simulink model "ps_model"  (R2025b)
settings: Solver=ode23tb  StartTime=0.0  StopTime=simlength  FixedStep=tc  MaxStep=tc
values from neighbouring files (symbols this model uses):
  omega_grid_emulator_nom = w_grid    (= 314.159265359)    [grid_emulator.m]
  omega_grid_nom = w_grid    (= 314.159265359)    [grid_emulator.m]
  ugrid_factor = 1    [grid_emulator.m]
  V_phase_normalization_factor = Vgrid_phase_normalization_factor    [grid_emulator.m]
  Vdc_base = 720    [grid_emulator.m]
  vn_eta_pu = 0    [grid_emulator.m]
  vn_xi_pu = 0    [grid_emulator.m]
  vp_xi_pu = 1    [grid_emulator.m]
undefined symbols (not defined in the file or in its folder): CFi, fnom, fPWM_INV, i_nom, ki_i, ki_u, kp_i, kp_u, Ld2_trafo_out, magnitude, n10, number_of_cells, omega_nom, Q, q1Kalman, q2Kalman, q3Kalman, R_RLload, Rd2_trafo_out, rKalman, tc, time_load_step, ts_afe, ts_inv, tsample, u_nom, Vdc_nom
libraries: fl_lib x120, nesl_utility x67, ee_lib x7, cstblocks x4, moving_average_filter x4, single_phase_transformer_lib x3, lithium_ion_cell_lib x1, simulink x1, threephase_inductor_lib x1
(part 2 of 4)

== system ps_model/inverter/3ph_Dyn_simscape ==
  Electrical Reference1 : fl_lib/Electrical/Electrical Elements/Electrical Reference
  ph1 : single_phase_transformer_lib/single phase transformer  Lm=Lmu2_trafo_out H  n1=sqrt(3)/0.8  n2=1  Rd1=Rd2_trafo_out/2 Ohm  Rd2=Rd2_trafo_out/2 Ohm  Ld1=Ld2_trafo_out/2 H  Ld2=Ld2_trafo_out/2 H  Rfe=Rm2_trafo_out Ohm  phi_specify=off  phi_priority=None  phi=0 V*s  phi_nominal_specify=off  phi_nominal_value=1  phi_nominal_unit=V*s  i1_specify=off  i1_priority=None  i1=0 A  i1_nominal_specify=off  i1_nominal_value=1  i1_nominal_unit=A  i2_specify=off  i2_priority=None  i2=0 A  i2_nominal_specify=off  i2_nominal_value=1  i2_nominal_unit=A  ife_specify=off  ife_priority=None  ife=0 A  ife_nominal_specify=off  ife_nominal_value=1  ife_nominal_unit=A  u1_specify=off  u1_priority=None  u1=0 V  u1_nominal_specify=off  u1_nominal_value=1  u1_nominal_unit=V  u2_specify=off  u2_priority=None  u2=0 V  u2_nominal_specify=off  u2_nominal_value=1  u2_nominal_unit=V
      settings: InternalSimscapePortConfiguration="{\"Bottom\":[],\"Left\":[{\"id\":\"u1_p\",\"label\":\"u1(+)\",\"type\":\"foundation.electrical.electrical\"},{\"id\":\"u1_n\",\"label\":\"u1(-)\",\"type\":\"foundation.electrical.electrical\"}],\"Right\":[{\"id\":\"u2_p\",\"label\":\"u2(+)\",\"type\":\"foundation.electrical.electrical\"},{\"id\":\"u2_n\",\"label\":\"u2(-)\",\"type\":\"foundation.electrical.electrical\"}],\"Top\":[]}"
  ph2 : single_phase_transformer_lib/single phase transformer  Lm=Lmu2_trafo_out H  n1=sqrt(3)/0.8  n2=1  Rd1=Rd2_trafo_out/2 Ohm  Rd2=Rd2_trafo_out/2 Ohm  Ld1=Ld2_trafo_out/2 H  Ld2=Ld2_trafo_out/2 H  Rfe=Rm2_trafo_out Ohm  phi_specify=off  phi_priority=None  phi=0 V*s  phi_nominal_specify=off  phi_nominal_value=1  phi_nominal_unit=V*s  i1_specify=off  i1_priority=None  i1=0 A  i1_nominal_specify=off  i1_nominal_value=1  i1_nominal_unit=A  i2_specify=off  i2_priority=None  i2=0 A  i2_nominal_specify=off  i2_nominal_value=1  i2_nominal_unit=A  ife_specify=off  ife_priority=None  ife=0 A  ife_nominal_specify=off  ife_nominal_value=1  ife_nominal_unit=A  u1_specify=off  u1_priority=None  u1=0 V  u1_nominal_specify=off  u1_nominal_value=1  u1_nominal_unit=V  u2_specify=off  u2_priority=None  u2=0 V  u2_nominal_specify=off  u2_nominal_value=1  u2_nominal_unit=V
      settings: InternalSimscapePortConfiguration="{\"Bottom\":[],\"Left\":[{\"id\":\"u1_p\",\"label\":\"u1(+)\",\"type\":\"foundation.electrical.electrical\"},{\"id\":\"u1_n\",\"label\":\"u1(-)\",\"type\":\"foundation.electrical.electrical\"}],\"Right\":[{\"id\":\"u2_p\",\"label\":\"u2(+)\",\"type\":\"foundation.electrical.electrical\"},{\"id\":\"u2_n\",\"label\":\"u2(-)\",\"type\":\"foundation.electrical.electrical\"}],\"Top\":[]}"
  ph3 : single_phase_transformer_lib/single phase transformer  Lm=Lmu2_trafo_out H  n1=sqrt(3)/0.8  n2=1  Rd1=Rd2_trafo_out/2 Ohm  Rd2=Rd2_trafo_out/2 Ohm  Ld1=Ld2_trafo_out/2 H  Ld2=Ld2_trafo_out/2 H  Rfe=Rm2_trafo_out Ohm  phi_specify=off  phi_priority=None  phi=0 V*s  phi_nominal_specify=off  phi_nominal_value=1  phi_nominal_unit=V*s  i1_specify=off  i1_priority=None  i1=0 A  i1_nominal_specify=off  i1_nominal_value=1  i1_nominal_unit=A  i2_specify=off  i2_priority=None  i2=0 A  i2_nominal_specify=off  i2_nominal_value=1  i2_nominal_unit=A  ife_specify=off  ife_priority=None  ife=0 A  ife_nominal_specify=off  ife_nominal_value=1  ife_nominal_unit=A  u1_specify=off  u1_priority=None  u1=0 V  u1_nominal_specify=off  u1_nominal_value=1  u1_nominal_unit=V  u2_specify=off  u2_priority=None  u2=0 V  u2_nominal_specify=off  u2_nominal_value=1  u2_nominal_unit=V
      settings: InternalSimscapePortConfiguration="{\"Bottom\":[],\"Left\":[{\"id\":\"u1_p\",\"label\":\"u1(+)\",\"type\":\"foundation.electrical.electrical\"},{\"id\":\"u1_n\",\"label\":\"u1(-)\",\"type\":\"foundation.electrical.electrical\"}],\"Right\":[{\"id\":\"u2_p\",\"label\":\"u2(+)\",\"type\":\"foundation.electrical.electrical\"},{\"id\":\"u2_n\",\"label\":\"u2(-)\",\"type\":\"foundation.electrical.electrical\"}],\"Top\":[]}"
  ua : PMIOPort  Side=Right
  ub : PMIOPort  Port=2  Side=Right
  uc : PMIOPort  Port=3  Side=Right
  Ua : PMIOPort  Port=4  Side=Left
  Ub : PMIOPort  Port=5  Side=Left
  Uc : PMIOPort  Port=6  Side=Left
  n : PMIOPort  Port=7  Side=Right
  connections:
  Electrical Reference1/LConn1 -- ph3/RConn2 -- ph2/RConn2 -- ph1/RConn2 -- n/RConn1
  ph3/RConn1 -- uc/RConn1
  ph1/RConn1 -- ua/RConn1
  ph2/RConn1 -- ub/RConn1
  Ua/RConn1 -- ph3/LConn2 -- ph1/LConn1
  ph1/LConn2 -- ph2/LConn1 -- Ub/RConn1
  Uc/RConn1 -- ph3/LConn1 -- ph2/LConn2

== system ps_model/inverter/LCL_filter ==
  CFu1 : fl_lib/Electrical/Electrical Elements/Capacitor  c=CFu F  r=RCFu Ohm  g=0 1/Ohm  i_specify=off  i_priority=None  i=0 A  i_nominal_specify=off  i_nominal_value=1  i_nominal_unit=A  v_specify=off  v_priority=None  v=0 V  v_nominal_specify=off  v_nominal_value=1  v_nominal_unit=V  vc_specify=off  vc_priority=High  vc=0 V  vc_nominal_specify=off  vc_nominal_value=1  vc_nominal_unit=V
  CFu2 : fl_lib/Electrical/Electrical Elements/Capacitor  c=CFu F  r=RCFu Ohm  g=0 1/Ohm  i_specify=off  i_priority=None  i=0 A  i_nominal_specify=off  i_nominal_value=1  i_nominal_unit=A  v_specify=off  v_priority=None  v=0 V  v_nominal_specify=off  v_nominal_value=1  v_nominal_unit=V  vc_specify=off  vc_priority=High  vc=0 V  vc_nominal_specify=off  vc_nominal_value=1  vc_nominal_unit=V
  CFu3 : fl_lib/Electrical/Electrical Elements/Capacitor  c=CFu F  r=RCFu Ohm  g=0 1/Ohm  i_specify=off  i_priority=None  i=0 A  i_nominal_specify=off  i_nominal_value=1  i_nominal_unit=A  v_specify=off  v_priority=None  v=0 V  v_nominal_specify=off  v_nominal_value=1  v_nominal_unit=V  vc_specify=off  vc_priority=High  vc=0 V  vc_nominal_specify=off  vc_nominal_value=1  vc_nominal_unit=V
  Current Sensor1 : fl_lib/Electrical/Electrical Sensors/Current Sensor
  Electrical Reference2 : fl_lib/Electrical/Electrical Elements/Electrical Reference
  Inductor : fl_lib/Electrical/Electrical Elements/Inductor  l=1e-6 H  r=0 Ohm  g=1e-9 1/Ohm  i_specify=on  i_priority=High  i=0 A  i_nominal_specify=off  i_nominal_value=1  i_nominal_unit=A  v_specify=off  v_priority=None  v=0 V  v_nominal_specify=off  v_nominal_value=1  v_nominal_unit=V  i_L_specify=off  i_L_priority=High  i_L=0 A  i_L_nominal_specify=off  i_L_nominal_value=1  i_L_nominal_unit=A
  Inductor1 : fl_lib/Electrical/Electrical Elements/Inductor  l=1e-6 H  r=0 Ohm  g=1e-9 1/Ohm  i_specify=on  i_priority=High  i=0 A  i_nominal_specify=off  i_nominal_value=1  i_nominal_unit=A  v_specify=off  v_priority=None  v=0 V  v_nominal_specify=off  v_nominal_value=1  v_nominal_unit=V  i_L_specify=off  i_L_priority=High  i_L=0 A  i_L_nominal_specify=off  i_L_nominal_value=1  i_L_nominal_unit=A
  Inductor2 : fl_lib/Electrical/Electrical Elements/Inductor  l=1e-6 H  r=0 Ohm  g=1e-9 1/Ohm  i_specify=on  i_priority=High  i=0 A  i_nominal_specify=off  i_nominal_value=1  i_nominal_unit=A  v_specify=off  v_priority=None  v=0 V  v_nominal_specify=off  v_nominal_value=1  v_nominal_unit=V  i_L_specify=off  i_L_priority=High  i_L=0 A  i_L_nominal_specify=off  i_L_nominal_value=1  i_L_nominal_unit=A
  iCFu : nesl_utility/PS-Simulink Converter  PhysicalDomain=network_engine_domain  SubClassName=ps_output  LeftPortType=input  RightPortType=output  PseudoPeriodic=off  Frequencies=[]  VectorFormat=1-D array  Unit=A  AffineConversion=off
  i_CFu : Scope
      settings: SampleTime=tc  ActiveDisplayYMinimum=-85.65604  ActiveDisplayYMaximum=85.78889
  threephase inductor : threephase_inductor_lib/threephase inductor  Lp=LFu1_AFE H  L0=LFu1_AFE_0 H  Rp=2.4e-3 Ohm  R0=0.8e-3 Ohm  Lls=5e-6 H  uu_1_specify=off  uu_1_priority=None  uu_1=0 V  uu_1_nominal_specify=off  uu_1_nominal_value=1  uu_1_nominal_unit=V  uv_1_specify=off  uv_1_priority=None  uv_1=0 V  uv_1_nominal_specify=off  uv_1_nominal_value=1  uv_1_nominal_unit=V  uw_1_specify=off  uw_1_priority=None  uw_1=0 V  uw_1_nominal_specify=off  uw_1_nominal_value=1  uw_1_nominal_unit=V  uu_2_specify=off  uu_2_priority=None  uu_2=0 V  uu_2_nominal_specify=off  uu_2_nominal_value=1  uu_2_nominal_unit=V  uv_2_specify=off  uv_2_priority=None  uv_2=0 V  uv_2_nominal_specify=off  uv_2_nominal_value=1  uv_2_nominal_unit=V  uw_2_specify=off  uw_2_priority=None  uw_2=0 V  uw_2_nominal_specify=off  uw_2_nominal_value=1  uw_2_nominal_unit=V  iu_specify=off  iu_priority=High  iu=0 A  iu_nominal_specify=off  iu_nominal_value=1  iu_nominal_unit=A  iv_specify=off  iv_priority=High  iv=0 A  iv_nominal_specify=off  iv_nominal_value=1  iv_nominal_unit=A  iw_specify=off  iw_priority=High  iw=0 A  iw_nominal_specify=off  iw_nominal_value=1  iw_nominal_unit=A
      settings: InternalSimscapePortConfiguration="{\"Bottom\":[],\"Left\":[{\"id\":\"up1\",\"label\":\"u1\",\"type\":\"foundation.electrical.electrical\"},{\"id\":\"vp1\",\"label\":\"v1\",\"type\":\"foundation.electrical.electrical\"},{\"id\":\"wp1\",\"label\":\"w1\",\"type\":\"foundation.electrical.electrical\"}],\"Right\":[{\"id\":\"up2\",\"label\":\"u2\",\"type\":\"foundation.electrical.electrical\"},{\"id\":\"vp2\",\"label\":\"v2\",\"type\":\"foundation.electrical.electrical\"},{\"id\":\"wp2\",\"label\":\"w2\",\"type\":\"foundation.electrical.electrical\"}],\"Top\":[]}"
  threephase_vi_measures_out1 : Subsystem
  threephase_vi_measures_stack : Subsystem
  us_a : PMIOPort  Side=Left
  uu : PMIOPort  Port=2  Side=Right
  us_b : PMIOPort  Port=3  Side=Left
  uv : PMIOPort  Port=4  Side=Right
  us_c : PMIOPort  Port=5  Side=Left
  uw : PMIOPort  Port=6  Side=Right
  output_filter_ct : PMIOPort  Port=7  Side=Right
  tag scope: i_CFu=global
  wires:
  iCFu/1 -> [i_CFu]  "i_cfu"
  [i_CFu] -> i_CFu/1
  connections:
  Inductor/RConn1 -- threephase_vi_measures_out1/LConn1 -- CFu1/LConn1
  Inductor2/RConn1 -- Current Sensor1/LConn1 -- threephase_vi_measures_out1/LConn3
  Inductor1/RConn1 -- threephase_vi_measures_out1/LConn2 -- CFu2/LConn1
  threephase_vi_measures_stack/LConn1 -- us_a/RConn1
  threephase_vi_measures_stack/LConn2 -- us_b/RConn1
  threephase_vi_measures_stack/LConn3 -- us_c/RConn1
  threephase_vi_measures_stack/RConn1 -- threephase inductor/LConn1
  threephase_vi_measures_stack/RConn2 -- threephase inductor/LConn2
  threephase_vi_measures_stack/RConn3 -- threephase inductor/LConn3
  threephase inductor/RConn1 -- Inductor/LConn1
  Inductor1/LConn1 -- threephase inductor/RConn2
  Inductor2/LConn1 -- threephase inductor/RConn3
  threephase_vi_measures_out1/RConn1 -- uu/RConn1
  threephase_vi_measures_out1/RConn2 -- uv/RConn1
  threephase_vi_measures_out1/RConn3 -- uw/RConn1
  Current Sensor1/RConn2 -- CFu3/LConn1
  Current Sensor1/RConn1 -- iCFu/LConn1
  CFu3/RConn1 -- output_filter_ct/RConn1 -- CFu2/RConn1 -- CFu1/RConn1

== system ps_model/inverter/MOS based inverter ==
  uab : Inport
  Constant1 : Constant
  Constant2 : Constant  Value=0
  Demux : Demux  Outputs=6
  inverter : Subsystem
  spwm : Subsystem  Commented=on
  sv_pwm : Subsystem
  u : PMIOPort  Side=Left
  v : PMIOPort  Port=2  Side=Left
  w : PMIOPort  Port=3  Side=Left
  udc(+) : PMIOPort  Port=4  Side=Right
  udc(-) : PMIOPort  Port=5  Side=Right
  tag scope: gm1=global, gm2=global, gm3=global, gm4=global, gm5=global, gm6=global
  wires:
  Demux/6 -> [gm6]
  Demux/4 -> [gm4]
  Demux/5 -> [gm5]
  Demux/3 -> [gm3]
  Demux/1 -> [gm1]
  Demux/2 -> [gm2]
  sv_pwm/1(cmd_gates) -> Demux/1
  uab/1 -> sv_pwm/1(ab)
  Constant2/1 -> sv_pwm/3(pwm_phase)
  Constant1/1 -> sv_pwm/2(enable)
  connections:
  inverter/LConn1 -- udc(+)/RConn1
  inverter/LConn2 -- udc(-)/RConn1
  v/RConn1 -- inverter/RConn2
  inverter/RConn1 -- u/RConn1
  inverter/RConn3 -- w/RConn1

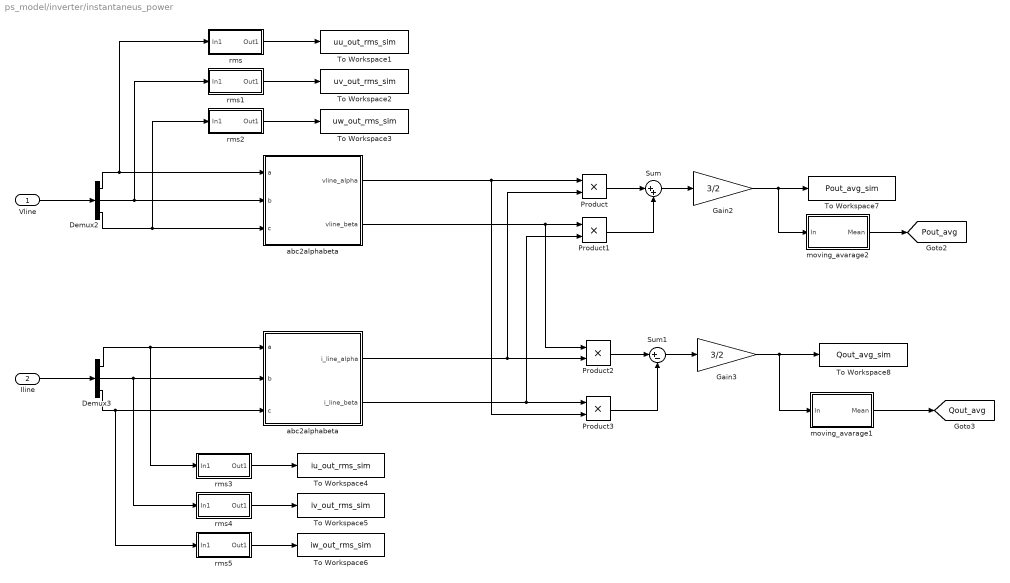
== system ps_model/inverter/instantaneus_power ==
  Vline : Inport
  Iline : Inport  Port=2
  Demux2 : Demux  Outputs=3
  Demux3 : Demux  Outputs=3
  Gain2 : Gain  Gain=3/2
  Gain3 : Gain  Gain=3/2
  Product{,1..3} (4 alike) : Product  RndMeth=Zero
  Sum : Sum  Inputs=|++
  Sum1 : Sum  Inputs=|+-
  To Workspace1 : ToWorkspace  VariableName=uu_out_rms_sim  SampleTime=ts_afe
      settings: MaxDataPoints=Ns_afe
  To Workspace2 : ToWorkspace  VariableName=uv_out_rms_sim  SampleTime=ts_afe
      settings: MaxDataPoints=Ns_afe
  To Workspace3 : ToWorkspace  VariableName=uw_out_rms_sim  SampleTime=ts_afe
      settings: MaxDataPoints=Ns_afe
  To Workspace4 : ToWorkspace  VariableName=iu_out_rms_sim  SampleTime=ts_afe
      settings: MaxDataPoints=Ns_afe
  To Workspace5 : ToWorkspace  VariableName=iv_out_rms_sim  SampleTime=ts_afe
      settings: MaxDataPoints=Ns_afe
  To Workspace6 : ToWorkspace  VariableName=iw_out_rms_sim  SampleTime=ts_afe
      settings: MaxDataPoints=Ns_afe
  To Workspace7 : ToWorkspace  VariableName=Pout_avg_sim  SampleTime=ts_afe
      settings: MaxDataPoints=Ns_afe
  To Workspace8 : ToWorkspace  VariableName=Qout_avg_sim  SampleTime=ts_afe
      settings: MaxDataPoints=Ns_afe
  abc2alphabeta : Subsystem
  "abc2alphabeta " : Subsystem
  moving_avarage1 : Subsystem
  moving_avarage2 : Subsystem
  rms : Subsystem
  rms1 : Subsystem
  rms2 : Subsystem
  rms3 : Subsystem
  rms4 : Subsystem
  rms5 : Subsystem
  tag scope: Pout_avg=global, Qout_avg=global
  wires:
  Gain3/1 -> moving_avarage1/1(In), To Workspace8/1
  Gain2/1 -> moving_avarage2/1(In), To Workspace7/1
  Demux2/1 -> rms/1(In1), abc2alphabeta/1(a)
  Vline/1 -> Demux2/1
  Iline/1 -> Demux3/1
  abc2alphabeta/2(vline_beta) -> Product1/1, Product2/1
  "abc2alphabeta "/2(i_line_beta) -> Product3/1, Product1/2
  abc2alphabeta/1(vline_alpha) -> Product/1, Product3/2
  "abc2alphabeta "/1(i_line_alpha) -> Product2/2, Product/2
  Product/1 -> Sum/1
  Product1/1 -> Sum/2
  Product2/1 -> Sum1/1
  Product3/1 -> Sum1/2
  Sum1/1 -> Gain3/1
  Sum/1 -> Gain2/1
  Demux2/2 -> rms1/1(In1), abc2alphabeta/2(b)
  Demux2/3 -> rms2/1(In1), abc2alphabeta/3(c)
  Demux3/1 -> "abc2alphabeta "/1(a), rms3/1(In1)
  Demux3/2 -> "abc2alphabeta "/2(b), rms4/1(In1)
  Demux3/3 -> rms5/1(In1), "abc2alphabeta "/3(c)
  moving_avarage2/1(Mean) -> [Pout_avg]
  moving_avarage1/1(Mean) -> [Qout_avg]
  rms/1(Out1) -> To Workspace1/1
  rms2/1(Out1) -> To Workspace3/1
  rms1/1(Out1) -> To Workspace2/1
  rms5/1(Out1) -> To Workspace6/1
  rms4/1(Out1) -> To Workspace5/1
  rms3/1(Out1) -> To Workspace4/1

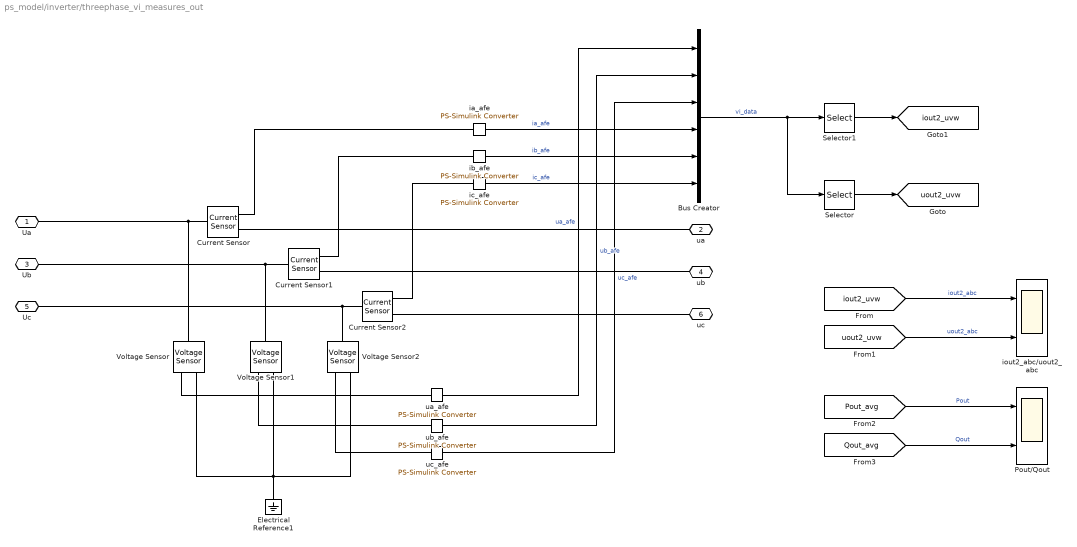
== system ps_model/inverter/threephase_vi_measures_out ==
  Bus Creator : BusCreator  Inputs=6
  Current Sensor : fl_lib/Electrical/Electrical Sensors/Current Sensor
  Current Sensor1 : fl_lib/Electrical/Electrical Sensors/Current Sensor
  Current Sensor2 : fl_lib/Electrical/Electrical Sensors/Current Sensor
  Electrical Reference1 : fl_lib/Electrical/Electrical Elements/Electrical Reference
  Pout/Qout : Scope  NumInputPorts=2
      settings: SampleTime=tc  ActiveDisplayYMinimum=-13623.318908223335  ActiveDisplayYMaximum=122609.87017401005  DataLoggingVariableName=ScopeData2
  Selector : Selector  InputPortWidth=6  IndexOptions=Index vector (dialog)  Indices=[1 2 3]  OutputSizes=1
  Selector1 : Selector  InputPortWidth=6  IndexOptions=Index vector (dialog)  Indices=[4 5 6]  OutputSizes=1
  Voltage Sensor : fl_lib/Electrical/Electrical Sensors/Voltage Sensor
  Voltage Sensor1 : fl_lib/Electrical/Electrical Sensors/Voltage Sensor
  Voltage Sensor2 : fl_lib/Electrical/Electrical Sensors/Voltage Sensor
  ia_afe : nesl_utility/PS-Simulink Converter  PhysicalDomain=network_engine_domain  SubClassName=ps_output  LeftPortType=input  RightPortType=output  PseudoPeriodic=off  Frequencies=[]  VectorFormat=1-D array  Unit=A  AffineConversion=off
  ib_afe : nesl_utility/PS-Simulink Converter  PhysicalDomain=network_engine_domain  SubClassName=ps_output  LeftPortType=input  RightPortType=output  PseudoPeriodic=off  Frequencies=[]  VectorFormat=1-D array  Unit=A  AffineConversion=off
  ic_afe : nesl_utility/PS-Simulink Converter  PhysicalDomain=network_engine_domain  SubClassName=ps_output  LeftPortType=input  RightPortType=output  PseudoPeriodic=off  Frequencies=[]  VectorFormat=1-D array  Unit=A  AffineConversion=off
  iout2_abc/uout2_abc : Scope  NumInputPorts=2
      settings: SampleTime=tc  ActiveDisplayYMinimum=-468.83601  ActiveDisplayYMaximum=470.63451
  ua_afe : nesl_utility/PS-Simulink Converter  PhysicalDomain=network_engine_domain  SubClassName=ps_output  LeftPortType=input  RightPortType=output  PseudoPeriodic=off  Frequencies=[]  VectorFormat=1-D array  Unit=V  AffineConversion=off
  ub_afe : nesl_utility/PS-Simulink Converter  PhysicalDomain=network_engine_domain  SubClassName=ps_output  LeftPortType=input  RightPortType=output  PseudoPeriodic=off  Frequencies=[]  VectorFormat=1-D array  Unit=V  AffineConversion=off
  uc_afe : nesl_utility/PS-Simulink Converter  PhysicalDomain=network_engine_domain  SubClassName=ps_output  LeftPortType=input  RightPortType=output  PseudoPeriodic=off  Frequencies=[]  VectorFormat=1-D array  Unit=V  AffineConversion=off
  Ua : PMIOPort  Side=Left
  ua : PMIOPort  Port=2  Side=Right
  Ub : PMIOPort  Port=3  Side=Left
  ub : PMIOPort  Port=4  Side=Right
  Uc : PMIOPort  Port=5  Side=Left
  uc : PMIOPort  Port=6  Side=Right
  tag scope: iout2_uvw=global, uout2_uvw=global
  wires:
  Bus Creator/1 -> Selector1/1, Selector/1  "vi_data"
  Selector/1 -> [uout2_uvw]
  ib_afe/1 -> Bus Creator/5  "ib_afe"
  ia_afe/1 -> Bus Creator/4  "ia_afe"
  ic_afe/1 -> Bus Creator/6  "ic_afe"
  ua_afe/1 -> Bus Creator/1  "ua_afe"
  ub_afe/1 -> Bus Creator/2  "ub_afe"
  uc_afe/1 -> Bus Creator/3  "uc_afe"
  Selector1/1 -> [iout2_uvw]
  [iout2_uvw] -> iout2_abc/uout2_abc/1  "iout2_abc"
  [uout2_uvw] -> iout2_abc/uout2_abc/2  "uout2_abc"
  [Pout_avg] -> Pout/Qout/1  "Pout"
  [Qout_avg] -> Pout/Qout/2  "Qout"
  connections:
  Current Sensor1/LConn1 -- Ub/RConn1 -- Voltage Sensor1/LConn1
  Electrical Reference1/LConn1 -- Voltage Sensor/RConn2 -- Voltage Sensor2/RConn2 -- Voltage Sensor1/RConn2
  Voltage Sensor/RConn1 -- ua_afe/LConn1
  Current Sensor/RConn2 -- ua/RConn1
  Voltage Sensor1/RConn1 -- ub_afe/LConn1
  Voltage Sensor2/LConn1 -- Uc/RConn1 -- Current Sensor2/LConn1
  Current Sensor/LConn1 -- Ua/RConn1 -- Voltage Sensor/LConn1
  Current Sensor1/RConn2 -- ub/RConn1
  Voltage Sensor2/RConn1 -- uc_afe/LConn1
  ib_afe/LConn1 -- Current Sensor1/RConn1
  ia_afe/LConn1 -- Current Sensor/RConn1
  ic_afe/LConn1 -- Current Sensor2/RConn1
  Current Sensor2/RConn2 -- uc/RConn1

== system ps_model/rectifier/rectifier ==
  Current Sensor1 : fl_lib/Electrical/Electrical Sensors/Current Sensor
  Diode{,1..5} (6 alike) : fl_lib/Electrical/Electrical Elements/Diode  Vf=Vgamma V  Ron=Ron Ohm  Goff=1e-8 1/Ohm  i_specify=off  i_priority=None  i=0 A  i_nominal_specify=off  i_nominal_value=1  i_nominal_unit=A  v_specify=off  v_priority=None  v=0 V  v_nominal_specify=off  v_nominal_value=1  v_nominal_unit=V
  Inductor : fl_lib/Electrical/Electrical Elements/Inductor  l=1e-6 H  r=0 Ohm  g=1e-3 1/Ohm  i_specify=off  i_priority=None  i=0 A  i_nominal_specify=off  i_nominal_value=1  i_nominal_unit=A  v_specify=off  v_priority=None  v=0 V  v_nominal_specify=off  v_nominal_value=1  v_nominal_unit=V  i_L_specify=off  i_L_priority=High  i_L=0 A  i_L_nominal_specify=off  i_L_nominal_value=1  i_L_nominal_unit=A
  Inductor1 : fl_lib/Electrical/Electrical Elements/Inductor  l=1e-6 H  r=0 Ohm  g=1e-3 1/Ohm  i_specify=off  i_priority=None  i=0 A  i_nominal_specify=off  i_nominal_value=1  i_nominal_unit=A  v_specify=off  v_priority=None  v=0 V  v_nominal_specify=off  v_nominal_value=1  v_nominal_unit=V  i_L_specify=off  i_L_priority=High  i_L=0 A  i_L_nominal_specify=off  i_L_nominal_value=1  i_L_nominal_unit=A
  Inductor2 : fl_lib/Electrical/Electrical Elements/Inductor  l=1e-6 H  r=0 Ohm  g=1e-3 1/Ohm  i_specify=off  i_priority=None  i=0 A  i_nominal_specify=off  i_nominal_value=1  i_nominal_unit=A  v_specify=off  v_priority=None  v=0 V  v_nominal_specify=off  v_nominal_value=1  v_nominal_unit=V  i_L_specify=off  i_L_priority=High  i_L=0 A  i_L_nominal_specify=off  i_L_nominal_value=1  i_L_nominal_unit=A
  Voltage Sensor2 : fl_lib/Electrical/Electrical Sensors/Voltage Sensor
  dclink_measure : Subsystem
  ileg_dc_inv : nesl_utility/PS-Simulink Converter  PhysicalDomain=network_engine_domain  SubClassName=ps_output  LeftPortType=input  RightPortType=output  PseudoPeriodic=off  Frequencies=[]  VectorFormat=1-D array  Unit=A  AffineConversion=on
  udc : nesl_utility/PS-Simulink Converter  PhysicalDomain=network_engine_domain  SubClassName=ps_output  LeftPortType=input  RightPortType=output  PseudoPeriodic=off  Frequencies=[]  VectorFormat=1-D array  Unit=V  AffineConversion=on
  us_a : PMIOPort  Side=Left
  us_b : PMIOPort  Port=2  Side=Left
  us_c : PMIOPort  Port=3  Side=Left
  Udc(+) : PMIOPort  Port=4  Side=Right
  Udc(-) : PMIOPort  Port=5  Side=Right
  tag scope: ileg_dc_afe_mod1=global, udc_mod1=global
  wires:
  udc/1 -> [udc_mod1]  "udc"
  ileg_dc_inv/1 -> [ileg_dc_afe_mod1]
  connections:
  Udc(+)/RConn1 -- Voltage Sensor2/LConn1 -- Current Sensor1/LConn1 -- Diode2/RConn1 -- Diode1/RConn1
  Udc(-)/RConn1 -- Voltage Sensor2/RConn2 -- Diode5/LConn1 -- Diode4/LConn1 -- Diode3/LConn1
  Inductor/LConn1 -- Diode5/RConn1 -- Diode/LConn1
  Inductor1/LConn1 -- Diode4/RConn1 -- Diode1/LConn1
  Inductor2/RConn1 -- us_c/RConn1
  Voltage Sensor2/RConn1 -- udc/LConn1 -- dclink_measure/LConn1
  Diode/RConn1 -- Current Sensor1/RConn2
  Current Sensor1/RConn1 -- ileg_dc_inv/LConn1
  Inductor/RConn1 -- us_a/RConn1
  Inductor1/RConn1 -- us_b/RConn1
  Inductor2/LConn1 -- Diode3/RConn1 -- Diode2/LConn1

== system ps_model/battery_system/battery_system/LithiumIonBattery ==
  Current Sensor : fl_lib/Electrical/Electrical Sensors/Current Sensor
  Electrical Reference1 : fl_lib/Electrical/Electrical Elements/Electrical Reference
  PS-Simulink Converter4 : nesl_utility/PS-Simulink Converter  PhysicalDomain=network_engine_domain  SubClassName=ps_output  LeftPortType=input  RightPortType=output  PseudoPeriodic=off  Frequencies=[]  VectorFormat=1-D array  Unit=1  AffineConversion=off
  PS-Simulink Converter5 : nesl_utility/PS-Simulink Converter  PhysicalDomain=network_engine_domain  SubClassName=ps_output  LeftPortType=input  RightPortType=output  PseudoPeriodic=off  Frequencies=[]  VectorFormat=1-D array  Unit=V  AffineConversion=on
  SOC_estimator : Subsystem
  To Workspace1 : ToWorkspace  VariableName=idc_battery_sim  SampleTime=tc
      settings: MaxDataPoints=Nc
  To Workspace2 : ToWorkspace  VariableName=udc_battery_sim  SampleTime=tc
      settings: MaxDataPoints=Nc
  Unit Delay5 : UnitDelay  SampleTime=tsample  HasFrameUpgradeWarning=on
  Voltage Sensor : fl_lib/Electrical/Electrical Sensors/Voltage Sensor
  ibat/vdc : Scope  Commented=on  NumInputPorts=2
      settings: SampleTime=tsample  ActiveDisplayYMinimum=-422.32966  ActiveDisplayYMaximum=499.01489  DataLoggingVariableName=ScopeData6
  lithium ion cell analytical ocv : Subsystem
  Uout+ : PMIOPort  Side=Right
  Uout- : PMIOPort  Port=2  Side=Right
  wires:
  PS-Simulink Converter5/1 -> Unit Delay5/1
  PS-Simulink Converter4/1 -> To Workspace1/1, ibat/vdc/1  "i batt"
  Unit Delay5/1 -> To Workspace2/1, [vdc]
  [vdc] -> ibat/vdc/2  "vdc"
  connections:
  Current Sensor/RConn1 -- PS-Simulink Converter4/LConn1
  Uout+/RConn1 -- Current Sensor/RConn2 -- Voltage Sensor/LConn1
  Voltage Sensor/RConn1 -- PS-Simulink Converter5/LConn1
  Voltage Sensor/RConn2 -- Electrical Reference1/LConn1 -- lithium ion cell analytical ocv/RConn2 -- Uout-/RConn1
  lithium ion cell analytical ocv/RConn1 -- Current Sensor/LConn1

== system ps_model/control_system/current_measure/current_transformation ==
  u : Inport
  v : Inport  Port=2
  w : Inport  Port=3
  phase : Inport  Port=4
  alphabeta2dq : MATLAB Function  TreatAsAtomicUnit=on  SystemSampleTime=ts_inv
  uvw2alphabeta : MATLAB Function  TreatAsAtomicUnit=on  SystemSampleTime=ts_inv
  tag scope: i_alpha_inverter_pu=global, i_beta_inverter_pu=global, id_inverter_pu=global, iq_inverter_pu=global
  wires:
  u/1 -> uvw2alphabeta/1(u)
  uvw2alphabeta/1(alpha) -> [i_alpha_inverter_pu], alphabeta2dq/1(alpha)  "ialpha_if_pu"
  uvw2alphabeta/2(beta) -> [i_beta_inverter_pu], alphabeta2dq/2(beta)  "ibeta_if_pu"
  v/1 -> uvw2alphabeta/2(v)
  w/1 -> uvw2alphabeta/3(w)
  alphabeta2dq/1(d) -> [id_inverter_pu]
  alphabeta2dq/2(q) -> [iq_inverter_pu]
  phase/1 -> alphabeta2dq/3(phase)

== system ps_model/control_system/current_measure/sample_hold_normalization ==
  iu : Inport
  iv : Inport  Port=2
  iw : Inport  Port=3
  Gain : Gain  Gain=1/i_nom
  Gain1 : Gain  Gain=1/i_nom
  Gain2 : Gain  Gain=1/i_nom
  Quantizer : Quantizer  QuantizationInterval=adc_quantizer
  Quantizer1 : Quantizer  QuantizationInterval=adc_quantizer
  Quantizer2 : Quantizer  QuantizationInterval=adc_quantizer
  Unit Delay : UnitDelay  SampleTime=ts_inv  HasFrameUpgradeWarning=on
  Unit Delay1 : UnitDelay  SampleTime=ts_inv  HasFrameUpgradeWarning=on
  Unit Delay4 : UnitDelay  SampleTime=ts_inv  HasFrameUpgradeWarning=on
  Zero-Order Hold : ZeroOrderHold  SampleTime=ts_inv
  Zero-Order Hold1 : ZeroOrderHold  SampleTime=ts_inv
  Zero-Order Hold2 : ZeroOrderHold  SampleTime=ts_inv
  iu_pu : Outport
  iv_pu : Outport  Port=2
  iw_pu : Outport  Port=3
  wires:
  Zero-Order Hold/1 -> Unit Delay/1
  Zero-Order Hold2/1 -> Unit Delay4/1
  Zero-Order Hold1/1 -> Unit Delay1/1
  Unit Delay1/1 -> iv_pu/1
  Unit Delay4/1 -> iw_pu/1
  Unit Delay/1 -> iu_pu/1
  iv/1 -> Gain1/1
  iu/1 -> Gain/1
  iw/1 -> Gain2/1
  Gain2/1 -> Quantizer2/1
  Gain1/1 -> Quantizer1/1
  Gain/1 -> Quantizer/1
  Quantizer/1 -> Zero-Order Hold/1
  Quantizer1/1 -> Zero-Order Hold1/1
  Quantizer2/1 -> Zero-Order Hold2/1

== system ps_model/control_system/scalar_voltage_control/pi_ctrl_i ==
  x : Inport
  xref : Inport  Port=2
  1/Ti : Gain  Gain=kp  SaturateOnIntegerOverflow=on  OutDataTypeStr=Inherit: Same as input  ParamDataTypeStr=Inherit: Same as input
  Saturation : Saturate  UpperLimit=sat_pos  LowerLimit=sat_neg
  Sum1 : Sum  Inputs=+++  SaturateOnIntegerOverflow=on
  Sum2 : Sum  Inputs=-+  SaturateOnIntegerOverflow=on
  Sum3 : Sum  Inputs=-+  SaturateOnIntegerOverflow=on
  Unit Delay4 : UnitDelay  SampleTime=ts  HasFrameUpgradeWarning=on
  kp : Gain  Gain=ki*ts  SaturateOnIntegerOverflow=on  OutDataTypeStr=Inherit: Same as input  ParamDataTypeStr=Inherit: Same as input
  u : Outport
  wires:
  xref/1 -> Sum2/2
  kp/1 -> Sum1/2
  Sum2/1 -> kp/1, 1/Ti/1
  1/Ti/1 -> Sum1/1, Sum3/1
  Sum3/1 -> Unit Delay4/1
  x/1 -> Sum2/1
  Sum1/1 -> Saturation/1
  Unit Delay4/1 -> Sum1/3
  Saturation/1 -> u/1, Sum3/2

== system ps_model/control_system/scalar_voltage_control/pi_ctrl_u ==
  x : Inport
  xref : Inport  Port=2
  1/Ti : Gain  Gain=kp  SaturateOnIntegerOverflow=on  OutDataTypeStr=Inherit: Same as input  ParamDataTypeStr=Inherit: Same as input
  Saturation : Saturate  UpperLimit=sat_pos  LowerLimit=sat_neg
  Sum1 : Sum  Inputs=+++  SaturateOnIntegerOverflow=on
  Sum2 : Sum  Inputs=-+  SaturateOnIntegerOverflow=on
  Sum3 : Sum  Inputs=-+  SaturateOnIntegerOverflow=on
  Unit Delay4 : UnitDelay  SampleTime=ts  HasFrameUpgradeWarning=on
  kp : Gain  Gain=ki*ts  SaturateOnIntegerOverflow=on  OutDataTypeStr=Inherit: Same as input  ParamDataTypeStr=Inherit: Same as input
  u : Outport
  wires:
  Saturation/1 -> Sum3/2, u/1
  Unit Delay4/1 -> Sum1/3
  Sum1/1 -> Saturation/1
  x/1 -> Sum2/1
  Sum3/1 -> Unit Delay4/1
  1/Ti/1 -> Sum3/1, Sum1/1
  Sum2/1 -> 1/Ti/1, kp/1
  kp/1 -> Sum1/2
  xref/1 -> Sum2/2

== system ps_model/control_system/voltage_measure/sample_hold_normalization ==
  iu : Inport
  iv : Inport  Port=2
  iw : Inport  Port=3
  Gain : Gain  Gain=1/u_nom
  Gain1 : Gain  Gain=1/u_nom
  Gain2 : Gain  Gain=1/u_nom
  Quantizer : Quantizer  QuantizationInterval=adc_quantizer
  Quantizer1 : Quantizer  QuantizationInterval=adc_quantizer
  Quantizer2 : Quantizer  QuantizationInterval=adc_quantizer
  Unit Delay : UnitDelay  SampleTime=ts_inv  HasFrameUpgradeWarning=on
  Unit Delay1 : UnitDelay  SampleTime=ts_inv  HasFrameUpgradeWarning=on
  Unit Delay4 : UnitDelay  SampleTime=ts_inv  HasFrameUpgradeWarning=on
  Zero-Order Hold : ZeroOrderHold  SampleTime=ts_inv
  Zero-Order Hold1 : ZeroOrderHold  SampleTime=ts_inv
  Zero-Order Hold2 : ZeroOrderHold  SampleTime=ts_inv
  uu_pu : Outport
  uv_pu : Outport  Port=2
  uw_pu : Outport  Port=3
  wires:
  iw/1 -> Gain2/1
  iu/1 -> Gain/1
  iv/1 -> Gain1/1
  Unit Delay/1 -> uu_pu/1
  Unit Delay4/1 -> uw_pu/1
  Unit Delay1/1 -> uv_pu/1
  Zero-Order Hold1/1 -> Unit Delay1/1
  Zero-Order Hold2/1 -> Unit Delay4/1
  Zero-Order Hold/1 -> Unit Delay/1
  Gain1/1 -> Quantizer1/1
  Gain/1 -> Quantizer/1
  Gain2/1 -> Quantizer2/1
  Quantizer/1 -> Zero-Order Hold/1
  Quantizer1/1 -> Zero-Order Hold1/1
  Quantizer2/1 -> Zero-Order Hold2/1

== system ps_model/control_system/voltage_measure/voltage_transformation ==
  u : Inport
  v : Inport  Port=2
  w : Inport  Port=3
  phase : Inport  Port=4
  alphabeta2dq : MATLAB Function  TreatAsAtomicUnit=on  SystemSampleTime=ts_inv
  uvw2alphabeta : MATLAB Function  TreatAsAtomicUnit=on  SystemSampleTime=ts_inv
  tag scope: u_alpha_out_pu=global, u_beta_out_pu=global, ud_out_pu=global, uq_out_pu=global
  wires:
  phase/1 -> alphabeta2dq/3(phase)
  w/1 -> uvw2alphabeta/3(w)
  v/1 -> uvw2alphabeta/2(v)
  uvw2alphabeta/2(beta) -> alphabeta2dq/2(beta), [u_beta_out_pu]  "ibeta_if_pu"
  uvw2alphabeta/1(alpha) -> alphabeta2dq/1(alpha), [u_alpha_out_pu]  "ialpha_if_pu"
  u/1 -> uvw2alphabeta/1(u)
  alphabeta2dq/1(d) -> [ud_out_pu]
  alphabeta2dq/2(q) -> [uq_out_pu]

== system ps_model/grid/grid_emulator/grid_emulator ==
  phase_gen : Subsystem
  voltage_reference : Subsystem
  voltage_source : Subsystem
  Vma : Outport
  Vmb : Outport  Port=2
  Vmc : Outport  Port=3
  wires:
  phase_gen/1(grid_emu_phase) -> voltage_reference/1(grid_emu_phase)  "grid_emu_phase"
  voltage_source/2(vn_xi) -> voltage_reference/3(Vxi_n)
  voltage_source/1(vp_xi) -> voltage_reference/2(Vxi_p)
  voltage_source/3(vn_eta) -> voltage_reference/4(Veta_n)
  voltage_reference/3(V3_ref) -> Vmc/1
  voltage_reference/1(V1_ref) -> Vma/1
  voltage_reference/2(V2_ref) -> Vmb/1

== system ps_model/grid/grid_emulator/threephase_vi_measures_mv ==
  Bus Creator : BusCreator  Inputs=6
  Current Sensor : fl_lib/Electrical/Electrical Sensors/Current Sensor
  Current Sensor1 : fl_lib/Electrical/Electrical Sensors/Current Sensor
  Current Sensor2 : fl_lib/Electrical/Electrical Sensors/Current Sensor
  Electrical Reference1 : fl_lib/Electrical/Electrical Elements/Electrical Reference
  Voltage Sensor : fl_lib/Electrical/Electrical Sensors/Voltage Sensor
  Voltage Sensor1 : fl_lib/Electrical/Electrical Sensors/Voltage Sensor
  Voltage Sensor2 : fl_lib/Electrical/Electrical Sensors/Voltage Sensor
  i : Selector  InputPortWidth=6  IndexOptions=Index vector (dialog)  Indices=[4 5 6]  OutputSizes=1
  i_line_abc/u_line_abc : Scope  NumInputPorts=2
      settings: SampleTime=tc  ActiveDisplayYMinimum=-3313.90419  ActiveDisplayYMaximum=3336.28901  DataLoggingVariableName=ScopeData2
  ia_grid : nesl_utility/PS-Simulink Converter  PhysicalDomain=network_engine_domain  SubClassName=ps_output  LeftPortType=input  RightPortType=output  PseudoPeriodic=off  Frequencies=[]  VectorFormat=1-D array  Unit=A  AffineConversion=off
  ib_grid : nesl_utility/PS-Simulink Converter  PhysicalDomain=network_engine_domain  SubClassName=ps_output  LeftPortType=input  RightPortType=output  PseudoPeriodic=off  Frequencies=[]  VectorFormat=1-D array  Unit=A  AffineConversion=off
  ic_grid : nesl_utility/PS-Simulink Converter  PhysicalDomain=network_engine_domain  SubClassName=ps_output  LeftPortType=input  RightPortType=output  PseudoPeriodic=off  Frequencies=[]  VectorFormat=1-D array  Unit=A  AffineConversion=off
  u : Selector  InputPortWidth=6  IndexOptions=Index vector (dialog)  Indices=[1 2 3]  OutputSizes=1
  ua_grid : nesl_utility/PS-Simulink Converter  PhysicalDomain=network_engine_domain  SubClassName=ps_output  LeftPortType=input  RightPortType=output  PseudoPeriodic=off  Frequencies=[]  VectorFormat=1-D array  Unit=V  AffineConversion=off
  ub_grid : nesl_utility/PS-Simulink Converter  PhysicalDomain=network_engine_domain  SubClassName=ps_output  LeftPortType=input  RightPortType=output  PseudoPeriodic=off  Frequencies=[]  VectorFormat=1-D array  Unit=V  AffineConversion=off
  uc_grid : nesl_utility/PS-Simulink Converter  PhysicalDomain=network_engine_domain  SubClassName=ps_output  LeftPortType=input  RightPortType=output  PseudoPeriodic=off  Frequencies=[]  VectorFormat=1-D array  Unit=V  AffineConversion=off
  Ua : PMIOPort  Side=Left
  ua : PMIOPort  Port=2  Side=Right
  Ub : PMIOPort  Port=3  Side=Left
  ub : PMIOPort  Port=4  Side=Right
  Uc : PMIOPort  Port=5  Side=Left
  uc : PMIOPort  Port=6  Side=Right
  wires:
  Bus Creator/1 -> i/1, u/1  "vi_data"
  ib_grid/1 -> Bus Creator/5  "ib"
  ia_grid/1 -> Bus Creator/4  "ia"
  ic_grid/1 -> Bus Creator/6  "ic"
  ua_grid/1 -> Bus Creator/1  "ua"
  ub_grid/1 -> Bus Creator/2  "ub"
  uc_grid/1 -> Bus Creator/3  "uc"
  i/1 -> i_line_abc/u_line_abc/1
  u/1 -> i_line_abc/u_line_abc/2
  connections:
  Current Sensor1/LConn1 -- Ub/RConn1 -- Voltage Sensor1/LConn1
  Electrical Reference1/LConn1 -- Voltage Sensor/RConn2 -- Voltage Sensor2/RConn2 -- Voltage Sensor1/RConn2
  Voltage Sensor/RConn1 -- ua_grid/LConn1
  Current Sensor/RConn2 -- ua/RConn1
  Voltage Sensor1/RConn1 -- ub_grid/LConn1
  Voltage Sensor2/LConn1 -- Current Sensor2/LConn1 -- Uc/RConn1
  Current Sensor/LConn1 -- Ua/RConn1 -- Voltage Sensor/LConn1
  Current Sensor1/RConn2 -- ub/RConn1
  Voltage Sensor2/RConn1 -- uc_grid/LConn1
  ib_grid/LConn1 -- Current Sensor1/RConn1
  ia_grid/LConn1 -- Current Sensor/RConn1
  ic_grid/LConn1 -- Current Sensor2/RConn1
  Current Sensor2/RConn2 -- uc/RConn1

== system ps_model/grid/instantaneus_power/abc2alphabeta ==
  a : Inport
  b : Inport  Port=2
  c : Inport  Port=3
  abc2alphabeta : Subsystem
  vline_alpha : Outport  VectorParamsAs1DForOutWhenUnconnected=off
  vline_beta : Outport  Port=2  VectorParamsAs1DForOutWhenUnconnected=off
  wires:
  a/1 -> abc2alphabeta/1(a)
  b/1 -> abc2alphabeta/2(b)
  c/1 -> abc2alphabeta/3(c)
  abc2alphabeta/2("beta ") -> vline_beta/1
  abc2alphabeta/1("alpha ") -> vline_alpha/1

== system ps_model/grid/instantaneus_power/abc2alphabeta  ==
  a : Inport
  b : Inport  Port=2
  c : Inport  Port=3
  abc->alphabeta : Subsystem
  i_line_alpha : Outport  VectorParamsAs1DForOutWhenUnconnected=off
  i_line_beta : Outport  Port=2  VectorParamsAs1DForOutWhenUnconnected=off
  wires:
  abc->alphabeta/1("alpha ") -> i_line_alpha/1
  abc->alphabeta/2("beta ") -> i_line_beta/1
  c/1 -> abc->alphabeta/3(c)
  b/1 -> abc->alphabeta/2(b)
  a/1 -> abc->alphabeta/1(a)

== system ps_model/grid/instantaneus_power/moving_avarage1 ==
  In : Inport
  Constant : Constant  Value=omega_grid_nom
  Zero-Order Hold : ZeroOrderHold  SampleTime=ts_afe
  dmavg_flt : moving_average_filter/dmavg_flt  ts=ts_afe  enable_time=0.025
  Mean : Outport  VectorParamsAs1DForOutWhenUnconnected=off
  wires:
  Zero-Order Hold/1 -> dmavg_flt/1
  In/1 -> Zero-Order Hold/1
  dmavg_flt/1 -> Mean/1
  Constant/1 -> dmavg_flt/2

== system ps_model/grid/instantaneus_power/moving_avarage2 ==
  In : Inport
  Constant : Constant  Value=omega_grid_nom
  Zero-Order Hold : ZeroOrderHold  SampleTime=ts_afe
  dmavg_flt : moving_average_filter/dmavg_flt  ts=ts_afe  enable_time=0.025
  Mean : Outport  VectorParamsAs1DForOutWhenUnconnected=off
  wires:
  Constant/1 -> dmavg_flt/2
  dmavg_flt/1 -> Mean/1
  In/1 -> Zero-Order Hold/1
  Zero-Order Hold/1 -> dmavg_flt/1

== system ps_model/grid/instantaneus_power/rms ==
  In1 : Inport
  Gain : Gain  Gain=n10-1
  Gain1 : Gain  Gain=1/n10
  Math Function : Math  Operator=magnitude^2  SignedPower=on
  Sqrt : Sqrt
  Sum : Sum  Inputs=|++
  Unit Delay : UnitDelay  SampleTime=ts_afe  HasFrameUpgradeWarning=on
  Out1 : Outport  VectorParamsAs1DForOutWhenUnconnected=off
  wires:
  In1/1 -> Math Function/1
  Sum/1 -> Gain1/1
  Gain1/1 -> Sqrt/1, Unit Delay/1
  Unit Delay/1 -> Gain/1
  Math Function/1 -> Sum/1
  Sqrt/1 -> Out1/1
  Gain/1 -> Sum/2

== system ps_model/grid/instantaneus_power/rms1 ==
  In1 : Inport
  Gain : Gain  Gain=n10-1
  Gain1 : Gain  Gain=1/n10
  Math Function : Math  Operator=magnitude^2  SignedPower=on
  Sqrt : Sqrt
  Sum : Sum  Inputs=|++
  Unit Delay : UnitDelay  SampleTime=ts_afe  HasFrameUpgradeWarning=on
  Out1 : Outport  VectorParamsAs1DForOutWhenUnconnected=off
  wires:
  Gain/1 -> Sum/2
  Sqrt/1 -> Out1/1
  Math Function/1 -> Sum/1
  Unit Delay/1 -> Gain/1
  Gain1/1 -> Unit Delay/1, Sqrt/1
  Sum/1 -> Gain1/1
  In1/1 -> Math Function/1

== system ps_model/grid/instantaneus_power/rms2 ==
  In1 : Inport
  Gain : Gain  Gain=n10-1
  Gain1 : Gain  Gain=1/n10
  Math Function : Math  Operator=magnitude^2  SignedPower=on
  Sqrt : Sqrt
  Sum : Sum  Inputs=|++
  Unit Delay : UnitDelay  SampleTime=ts_afe  HasFrameUpgradeWarning=on
  Out1 : Outport  VectorParamsAs1DForOutWhenUnconnected=off
  wires:
  In1/1 -> Math Function/1
  Sum/1 -> Gain1/1
  Gain1/1 -> Sqrt/1, Unit Delay/1
  Unit Delay/1 -> Gain/1
  Math Function/1 -> Sum/1
  Sqrt/1 -> Out1/1
  Gain/1 -> Sum/2

== system ps_model/grid/instantaneus_power/rms3 ==
  In1 : Inport
  Gain : Gain  Gain=n10-1
  Gain1 : Gain  Gain=1/n10
  Math Function : Math  Operator=magnitude^2  SignedPower=on
  Sqrt : Sqrt
  Sum : Sum  Inputs=|++
  Unit Delay : UnitDelay  SampleTime=ts_afe  HasFrameUpgradeWarning=on
  Out1 : Outport  VectorParamsAs1DForOutWhenUnconnected=off
  wires:
  Gain/1 -> Sum/2
  Sqrt/1 -> Out1/1
  Math Function/1 -> Sum/1
  Unit Delay/1 -> Gain/1
  Gain1/1 -> Unit Delay/1, Sqrt/1
  Sum/1 -> Gain1/1
  In1/1 -> Math Function/1

== system ps_model/grid/instantaneus_power/rms4 ==
  In1 : Inport
  Gain : Gain  Gain=n10-1
  Gain1 : Gain  Gain=1/n10
  Math Function : Math  Operator=magnitude^2  SignedPower=on
  Sqrt : Sqrt
  Sum : Sum  Inputs=|++
  Unit Delay : UnitDelay  SampleTime=ts_afe  HasFrameUpgradeWarning=on
  Out1 : Outport  VectorParamsAs1DForOutWhenUnconnected=off
  wires:
  In1/1 -> Math Function/1
  Sum/1 -> Gain1/1
  Gain1/1 -> Sqrt/1, Unit Delay/1
  Unit Delay/1 -> Gain/1
  Math Function/1 -> Sum/1
  Sqrt/1 -> Out1/1
  Gain/1 -> Sum/2

== system ps_model/grid/instantaneus_power/rms5 ==
  In1 : Inport
  Gain : Gain  Gain=n10-1
  Gain1 : Gain  Gain=1/n10
  Math Function : Math  Operator=magnitude^2  SignedPower=on
  Sqrt : Sqrt
  Sum : Sum  Inputs=|++
  Unit Delay : UnitDelay  SampleTime=ts_afe  HasFrameUpgradeWarning=on
  Out1 : Outport  VectorParamsAs1DForOutWhenUnconnected=off
  wires:
  Gain/1 -> Sum/2
  Sqrt/1 -> Out1/1
  Math Function/1 -> Sum/1
  Unit Delay/1 -> Gain/1
  Gain1/1 -> Unit Delay/1, Sqrt/1
  Sum/1 -> Gain1/1
  In1/1 -> Math Function/1

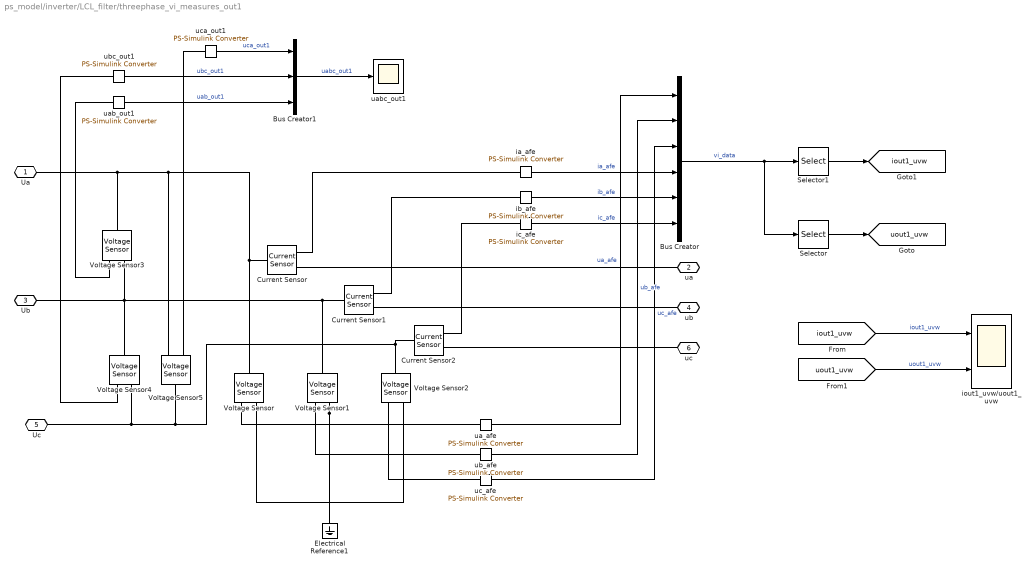
== system ps_model/inverter/LCL_filter/threephase_vi_measures_out1 ==
  Bus Creator : BusCreator  Inputs=6
  Bus Creator1 : BusCreator  Inputs=3
  Current Sensor : fl_lib/Electrical/Electrical Sensors/Current Sensor
  Current Sensor1 : fl_lib/Electrical/Electrical Sensors/Current Sensor
  Current Sensor2 : fl_lib/Electrical/Electrical Sensors/Current Sensor
  Electrical Reference1 : fl_lib/Electrical/Electrical Elements/Electrical Reference
  Selector : Selector  InputPortWidth=6  IndexOptions=Index vector (dialog)  Indices=[1 2 3]  OutputSizes=1
  Selector1 : Selector  InputPortWidth=6  IndexOptions=Index vector (dialog)  Indices=[4 5 6]  OutputSizes=1
  Voltage Sensor{,1..5} (6 alike) : fl_lib/Electrical/Electrical Sensors/Voltage Sensor
  ia_afe : nesl_utility/PS-Simulink Converter  PhysicalDomain=network_engine_domain  SubClassName=ps_output  LeftPortType=input  RightPortType=output  PseudoPeriodic=off  Frequencies=[]  VectorFormat=1-D array  Unit=A  AffineConversion=off
  ib_afe : nesl_utility/PS-Simulink Converter  PhysicalDomain=network_engine_domain  SubClassName=ps_output  LeftPortType=input  RightPortType=output  PseudoPeriodic=off  Frequencies=[]  VectorFormat=1-D array  Unit=A  AffineConversion=off
  ic_afe : nesl_utility/PS-Simulink Converter  PhysicalDomain=network_engine_domain  SubClassName=ps_output  LeftPortType=input  RightPortType=output  PseudoPeriodic=off  Frequencies=[]  VectorFormat=1-D array  Unit=A  AffineConversion=off
  iout1_uvw/uout1_uvw : Scope  NumInputPorts=2
      settings: SampleTime=tc  ActiveDisplayYMinimum=-157.88233  ActiveDisplayYMaximum=156.01454
  ua_afe : nesl_utility/PS-Simulink Converter  PhysicalDomain=network_engine_domain  SubClassName=ps_output  LeftPortType=input  RightPortType=output  PseudoPeriodic=off  Frequencies=[]  VectorFormat=1-D array  Unit=V  AffineConversion=off
  uab_out1 : nesl_utility/PS-Simulink Converter  PhysicalDomain=network_engine_domain  SubClassName=ps_output  LeftPortType=input  RightPortType=output  PseudoPeriodic=off  Frequencies=[]  VectorFormat=1-D array  Unit=V  AffineConversion=off
  uabc_out1 : Scope
      settings: SampleTime=tc  ActiveDisplayYMinimum=-470.50897  ActiveDisplayYMaximum=488.34757
  ub_afe : nesl_utility/PS-Simulink Converter  PhysicalDomain=network_engine_domain  SubClassName=ps_output  LeftPortType=input  RightPortType=output  PseudoPeriodic=off  Frequencies=[]  VectorFormat=1-D array  Unit=V  AffineConversion=off
  ubc_out1 : nesl_utility/PS-Simulink Converter  PhysicalDomain=network_engine_domain  SubClassName=ps_output  LeftPortType=input  RightPortType=output  PseudoPeriodic=off  Frequencies=[]  VectorFormat=1-D array  Unit=V  AffineConversion=off
  uc_afe : nesl_utility/PS-Simulink Converter  PhysicalDomain=network_engine_domain  SubClassName=ps_output  LeftPortType=input  RightPortType=output  PseudoPeriodic=off  Frequencies=[]  VectorFormat=1-D array  Unit=V  AffineConversion=off
  uca_out1 : nesl_utility/PS-Simulink Converter  PhysicalDomain=network_engine_domain  SubClassName=ps_output  LeftPortType=input  RightPortType=output  PseudoPeriodic=off  Frequencies=[]  VectorFormat=1-D array  Unit=V  AffineConversion=off
  Ua : PMIOPort  Side=Left
  ua : PMIOPort  Port=2  Side=Right
  Ub : PMIOPort  Port=3  Side=Left
  ub : PMIOPort  Port=4  Side=Right
  Uc : PMIOPort  Port=5  Side=Left
  uc : PMIOPort  Port=6  Side=Right
  tag scope: iout1_uvw=global, uout1_uvw=global
  wires:
  [uout1_uvw] -> iout1_uvw/uout1_uvw/2  "uout1_uvw"
  [iout1_uvw] -> iout1_uvw/uout1_uvw/1  "iout1_uvw"
  Selector1/1 -> [iout1_uvw]
  uc_afe/1 -> Bus Creator/3  "uc_afe"
  ub_afe/1 -> Bus Creator/2  "ub_afe"
  ua_afe/1 -> Bus Creator/1  "ua_afe"
  ic_afe/1 -> Bus Creator/6  "ic_afe"
  ia_afe/1 -> Bus Creator/4  "ia_afe"
  ib_afe/1 -> Bus Creator/5  "ib_afe"
  Selector/1 -> [uout1_uvw]
  Bus Creator/1 -> Selector/1, Selector1/1  "vi_data"
  uca_out1/1 -> Bus Creator1/1  "uca_out1"
  ubc_out1/1 -> Bus Creator1/2  "ubc_out1"
  uab_out1/1 -> Bus Creator1/3  "uab_out1"
  Bus Creator1/1 -> uabc_out1/1  "uabc_out1"
  connections:
  Current Sensor2/RConn2 -- uc/RConn1
  ic_afe/LConn1 -- Current Sensor2/RConn1
  ia_afe/LConn1 -- Current Sensor/RConn1
  ib_afe/LConn1 -- Current Sensor1/RConn1
  Voltage Sensor2/RConn1 -- uc_afe/LConn1
  Current Sensor1/RConn2 -- ub/RConn1
  Voltage Sensor/LConn1 -- Voltage Sensor5/RConn2 -- Voltage Sensor3/LConn1 -- Ua/RConn1 -- Current Sensor/LConn1
  Current Sensor2/LConn1 -- Voltage Sensor2/LConn1 -- Voltage Sensor5/LConn1 -- Voltage Sensor4/RConn2 -- Uc/RConn1
  Voltage Sensor1/RConn1 -- ub_afe/LConn1
  Current Sensor/RConn2 -- ua/RConn1
  Voltage Sensor/RConn1 -- ua_afe/LConn1
  Voltage Sensor1/RConn2 -- Voltage Sensor2/RConn2 -- Voltage Sensor/RConn2 -- Electrical Reference1/LConn1
  Voltage Sensor1/LConn1 -- Voltage Sensor3/RConn2 -- Voltage Sensor4/LConn1 -- Ub/RConn1 -- Current Sensor1/LConn1
  Voltage Sensor3/RConn1 -- uab_out1/LConn1
  ubc_out1/LConn1 -- Voltage Sensor4/RConn1
  uca_out1/LConn1 -- Voltage Sensor5/RConn1

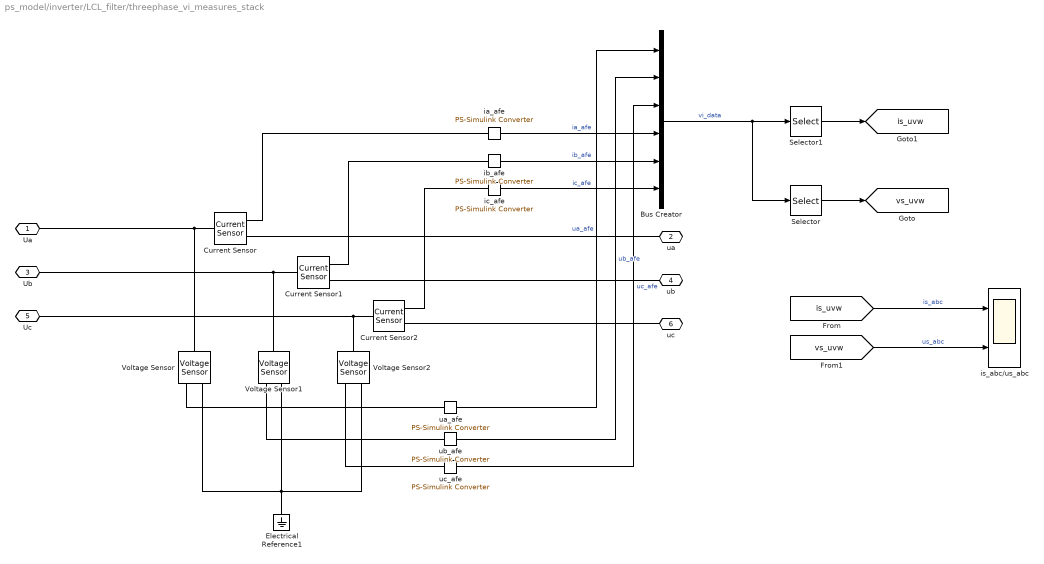
== system ps_model/inverter/LCL_filter/threephase_vi_measures_stack ==
  Bus Creator : BusCreator  Inputs=6
  Current Sensor : fl_lib/Electrical/Electrical Sensors/Current Sensor
  Current Sensor1 : fl_lib/Electrical/Electrical Sensors/Current Sensor
  Current Sensor2 : fl_lib/Electrical/Electrical Sensors/Current Sensor
  Electrical Reference1 : fl_lib/Electrical/Electrical Elements/Electrical Reference
  Selector : Selector  InputPortWidth=6  IndexOptions=Index vector (dialog)  Indices=[1 2 3]  OutputSizes=1
  Selector1 : Selector  InputPortWidth=6  IndexOptions=Index vector (dialog)  Indices=[4 5 6]  OutputSizes=1
  Voltage Sensor : fl_lib/Electrical/Electrical Sensors/Voltage Sensor
  Voltage Sensor1 : fl_lib/Electrical/Electrical Sensors/Voltage Sensor
  Voltage Sensor2 : fl_lib/Electrical/Electrical Sensors/Voltage Sensor
  ia_afe : nesl_utility/PS-Simulink Converter  PhysicalDomain=network_engine_domain  SubClassName=ps_output  LeftPortType=input  RightPortType=output  PseudoPeriodic=off  Frequencies=[]  VectorFormat=1-D array  Unit=A  AffineConversion=off
  ib_afe : nesl_utility/PS-Simulink Converter  PhysicalDomain=network_engine_domain  SubClassName=ps_output  LeftPortType=input  RightPortType=output  PseudoPeriodic=off  Frequencies=[]  VectorFormat=1-D array  Unit=A  AffineConversion=off
  ic_afe : nesl_utility/PS-Simulink Converter  PhysicalDomain=network_engine_domain  SubClassName=ps_output  LeftPortType=input  RightPortType=output  PseudoPeriodic=off  Frequencies=[]  VectorFormat=1-D array  Unit=A  AffineConversion=off
  is_abc/us_abc : Scope  NumInputPorts=2
      settings: SampleTime=tc  ActiveDisplayYMinimum=-384.2584  ActiveDisplayYMaximum=377.23948
  ua_afe : nesl_utility/PS-Simulink Converter  PhysicalDomain=network_engine_domain  SubClassName=ps_output  LeftPortType=input  RightPortType=output  PseudoPeriodic=off  Frequencies=[]  VectorFormat=1-D array  Unit=V  AffineConversion=off
  ub_afe : nesl_utility/PS-Simulink Converter  PhysicalDomain=network_engine_domain  SubClassName=ps_output  LeftPortType=input  RightPortType=output  PseudoPeriodic=off  Frequencies=[]  VectorFormat=1-D array  Unit=V  AffineConversion=off
  uc_afe : nesl_utility/PS-Simulink Converter  PhysicalDomain=network_engine_domain  SubClassName=ps_output  LeftPortType=input  RightPortType=output  PseudoPeriodic=off  Frequencies=[]  VectorFormat=1-D array  Unit=V  AffineConversion=off
  Ua : PMIOPort  Side=Left
  ua : PMIOPort  Port=2  Side=Right
  Ub : PMIOPort  Port=3  Side=Left
  ub : PMIOPort  Port=4  Side=Right
  Uc : PMIOPort  Port=5  Side=Left
  uc : PMIOPort  Port=6  Side=Right
  tag scope: is_uvw=global, vs_uvw=global
  wires:
  Bus Creator/1 -> Selector1/1, Selector/1  "vi_data"
  Selector/1 -> [vs_uvw]
  ib_afe/1 -> Bus Creator/5  "ib_afe"
  ia_afe/1 -> Bus Creator/4  "ia_afe"
  ic_afe/1 -> Bus Creator/6  "ic_afe"
  ua_afe/1 -> Bus Creator/1  "ua_afe"
  ub_afe/1 -> Bus Creator/2  "ub_afe"
  uc_afe/1 -> Bus Creator/3  "uc_afe"
  Selector1/1 -> [is_uvw]
  [is_uvw] -> is_abc/us_abc/1  "is_abc"
  [vs_uvw] -> is_abc/us_abc/2  "us_abc"
  connections:
  Current Sensor1/LConn1 -- Ub/RConn1 -- Voltage Sensor1/LConn1
  Electrical Reference1/LConn1 -- Voltage Sensor/RConn2 -- Voltage Sensor2/RConn2 -- Voltage Sensor1/RConn2
  Voltage Sensor/RConn1 -- ua_afe/LConn1
  Current Sensor/RConn2 -- ua/RConn1
  Voltage Sensor1/RConn1 -- ub_afe/LConn1
  Voltage Sensor2/LConn1 -- Uc/RConn1 -- Current Sensor2/LConn1
  Current Sensor/LConn1 -- Ua/RConn1 -- Voltage Sensor/LConn1
  Current Sensor1/RConn2 -- ub/RConn1
  Voltage Sensor2/RConn1 -- uc_afe/LConn1
  ib_afe/LConn1 -- Current Sensor1/RConn1
  ia_afe/LConn1 -- Current Sensor/RConn1
  ic_afe/LConn1 -- Current Sensor2/RConn1
  Current Sensor2/RConn2 -- uc/RConn1
